simulink model "SPWM"  (R2022a)
settings: Solver=ode23  StartTime=0.0  StopTime=0.05  MaxStep=1e-5  RelTol=1e-3
libraries: simulink x2, spspowerguiLib x1
settings Model: Creator=123  LastModifiedBy=123

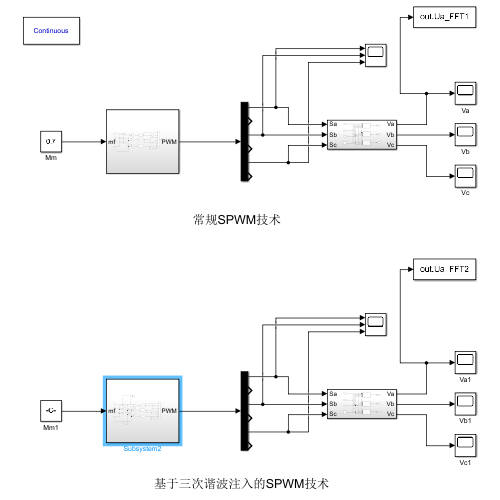
[thumbnail: Simulink's stored preview of the top-level diagram]
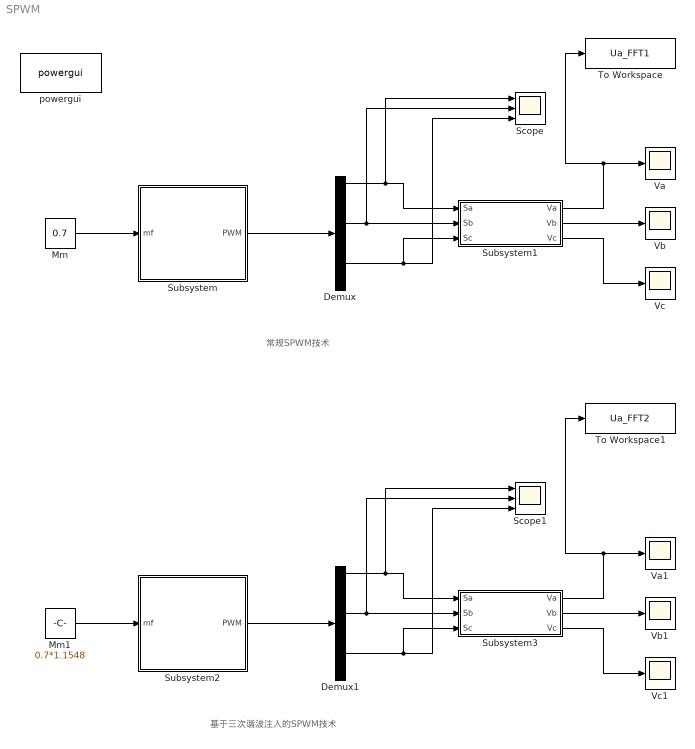
== system SPWM ==
  note: 基于三次谐波注入的SPWM技术
  note: 常规SPWM技术
  Demux : Demux  Outputs=6
  Demux1 : Demux  Outputs=6
  Mm : Constant  Value=0.7
  Mm1 : Constant  Value=0.7*1.1548
  Scope : Scope  NumInputPorts=3
  Scope1 : Scope  NumInputPorts=3
  Subsystem : Subsystem
  Subsystem1 : Subsystem
  Subsystem2 : Subsystem
  Subsystem3 : Subsystem
  To Workspace : ToWorkspace  VariableName=Ua_FFT1  SaveFormat=Structure With Time  SampleTime=1e-6
  To Workspace1 : ToWorkspace  VariableName=Ua_FFT2  SaveFormat=Structure With Time  SampleTime=1e-6
  Va : Scope
  Va1 : Scope
  Vb : Scope
  Vb1 : Scope
  Vc : Scope
  Vc1 : Scope
  powergui : spspowerguiLib/powergui  Priority=1  SimulationMode=Continuous  SampleTime=50e-6  frequency=60  Iterations=50  frequencyindice=60  Pbase=100e6  ErrMax=1e-4  UnitsV=kV  UnitsW=MW  buscounter=0  FunctionMessages=off  echomessages=off  EnableUseOfTLC=off  CurrentSourceSwitches=off  DisableSnubberDevices=off  DisableRonSwitches=off  DisableVfSwitches=off  DisplayEquations=off  AutomaticDiscreteSolvers=off  SolverType=Tustin/Backward Euler (TBE)  Interpol=off  ExternalGateDelay=off  methode=off  Ts=100  x0status=blocks  SPID=on  SwTol=0  HookPort=off  NonlinearTolerance=1e-4  nMaxIteration=100  ContinueOnMaxIteration=off  RestoreLinks=warning  ResistiveCurrentMeasurement=off  Frange=[0:2:500]  Ylog=off  Xlog=on  ShowGrid=off  save=off  variable=ZData  structure=0  ZoomFFT=off  StartTime=0.0  cycles=1  DisplayStyle=1  fundamental=60  FreqAxis=off  MaxFrequency=1000  frequencyindicesteady=1  RmsSteady=1  display=off
  wires:
  Mm/1 -> Subsystem/1(mf)
  Subsystem/1(PWM) -> Demux/1
  Demux/1 -> Scope/1, Subsystem1/1(Sa)
  Demux/3 -> Scope/2, Subsystem1/2(Sb)
  Demux/5 -> Scope/3, Subsystem1/3(Sc)
  Subsystem1/1(Va) -> Va/1, To Workspace/1
  Subsystem1/2(Vb) -> Vb/1
  Subsystem1/3(Vc) -> Vc/1
  Mm1/1 -> Subsystem2/1(mf)
  Subsystem2/1(PWM) -> Demux1/1
  Subsystem3/1(Va) -> Va1/1, To Workspace1/1
  Demux1/5 -> Scope1/3, Subsystem3/3(Sc)
  Subsystem3/3(Vc) -> Vc1/1
  Demux1/3 -> Scope1/2, Subsystem3/2(Sb)
  Subsystem3/2(Vb) -> Vb1/1
  Demux1/1 -> Scope1/1, Subsystem3/1(Sa)

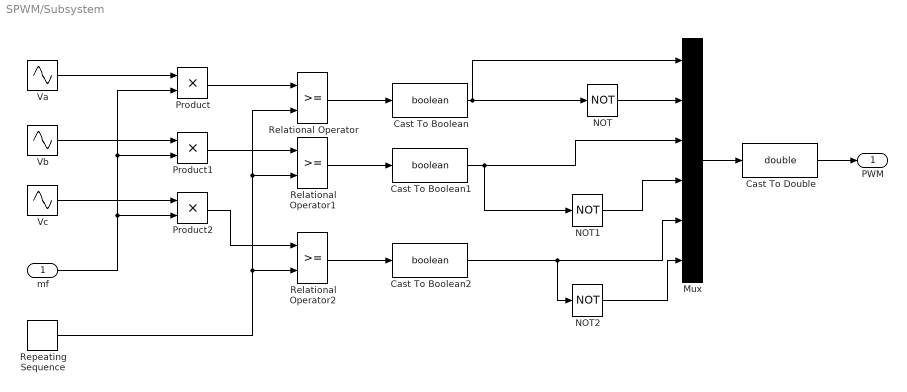
== system SPWM/Subsystem ==
  mf : Inport
  Cast To Boolean : DataTypeConversion  OutDataTypeStr=boolean  SaturateOnIntegerOverflow=off  RndMeth=Floor
  Cast To Boolean1 : DataTypeConversion  OutDataTypeStr=boolean  SaturateOnIntegerOverflow=off  RndMeth=Floor
  Cast To Boolean2 : DataTypeConversion  OutDataTypeStr=boolean  SaturateOnIntegerOverflow=off  RndMeth=Floor
  Cast To Double : DataTypeConversion  OutDataTypeStr=double  SaturateOnIntegerOverflow=off  RndMeth=Floor
  Mux : Mux  Inputs=6
  NOT : Logic  Operator=NOT  AllPortsSameDT=off  OutDataTypeStr=boolean
  NOT1 : Logic  Operator=NOT  AllPortsSameDT=off  OutDataTypeStr=boolean
  NOT2 : Logic  Operator=NOT  AllPortsSameDT=off  OutDataTypeStr=boolean
  Product : Product
  Product1 : Product
  Product2 : Product
  Relational Operator : RelationalOperator  OutDataTypeStr=boolean  RndMeth=Simplest  InputSameDT=off
  Relational Operator1 : RelationalOperator  OutDataTypeStr=boolean  RndMeth=Simplest  InputSameDT=off
  Relational Operator2 : RelationalOperator  OutDataTypeStr=boolean  RndMeth=Simplest  InputSameDT=off
  Repeating Sequence : simulink/Sources/Repeating Sequence  rep_seq_t=[0 0.00005 0.00015 0.0002]  rep_seq_y=[0 -1 1 0]
  Va : Sin  Frequency=2*50*pi  SampleTime=0
  Vb : Sin  Frequency=2*50*pi  Phase=-2/3*pi  SampleTime=0
  Vc : Sin  Frequency=2*50*pi  Phase=2/3*pi  SampleTime=0
  PWM : Outport
  wires:
  Va/1 -> Product/1
  mf/1 -> Product2/2, Product1/2, Product/2
  Vb/1 -> Product1/1
  Vc/1 -> Product2/1
  Product/1 -> Relational Operator/1
  Repeating Sequence/1 -> Relational Operator2/2, Relational Operator1/2, Relational Operator/2
  Product1/1 -> Relational Operator1/1
  Product2/1 -> Relational Operator2/1
  Relational Operator/1 -> Cast To Boolean/1
  Relational Operator2/1 -> Cast To Boolean2/1
  Relational Operator1/1 -> Cast To Boolean1/1
  Mux/1 -> Cast To Double/1
  Cast To Double/1 -> PWM/1
  Cast To Boolean/1 -> NOT/1, Mux/1
  NOT/1 -> Mux/2
  Cast To Boolean1/1 -> NOT1/1, Mux/3
  NOT1/1 -> Mux/4
  Cast To Boolean2/1 -> NOT2/1, Mux/5
  NOT2/1 -> Mux/6

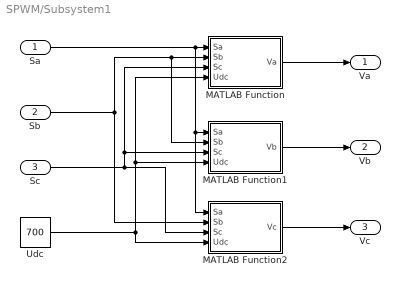
== system SPWM/Subsystem1 ==
  Sa : Inport
  Sb : Inport  Port=2
  Sc : Inport  Port=3
  MATLAB Function : MATLAB Function  TreatAsAtomicUnit=on
  MATLAB Function1 : MATLAB Function  TreatAsAtomicUnit=on
  MATLAB Function2 : MATLAB Function  TreatAsAtomicUnit=on
  Udc : Constant  Value=700
  Va : Outport
  Vb : Outport  Port=2
  Vc : Outport  Port=3
  wires:
  Sa/1 -> MATLAB Function1/1(Sa), MATLAB Function2/1(Sa), MATLAB Function/1(Sa)
  Sb/1 -> MATLAB Function2/2(Sb), MATLAB Function/2(Sb), MATLAB Function1/2(Sb)
  Sc/1 -> MATLAB Function2/3(Sc), MATLAB Function1/3(Sc), MATLAB Function/3(Sc)
  Udc/1 -> MATLAB Function2/4(Udc), MATLAB Function1/4(Udc), MATLAB Function/4(Udc)
  MATLAB Function2/1(Vc) -> Vc/1
  MATLAB Function1/1(Vb) -> Vb/1
  MATLAB Function/1(Va) -> Va/1

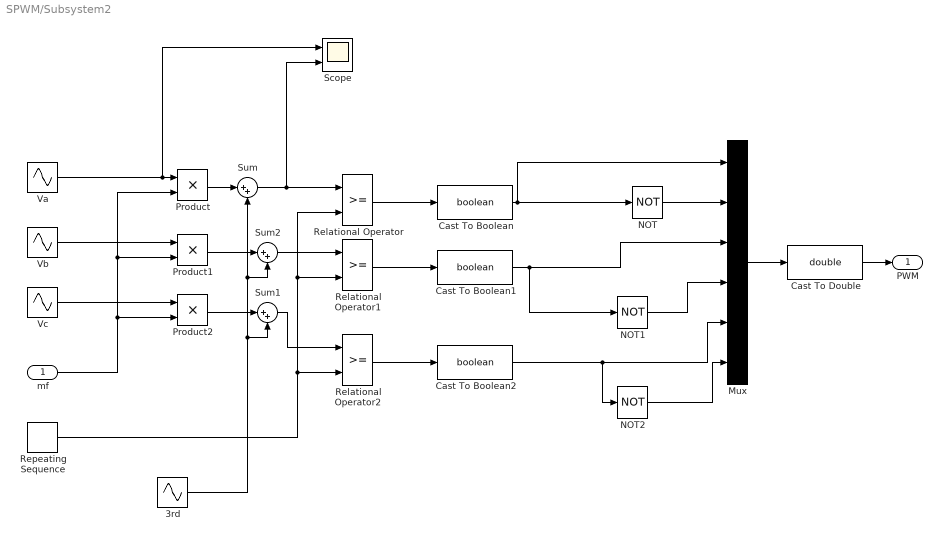
== system SPWM/Subsystem2 ==
  mf : Inport
  3rd : Sin  Amplitude=1*0.7*1.1548/6  Frequency=2*50*pi*3  SampleTime=0
  Cast To Boolean : DataTypeConversion  OutDataTypeStr=boolean  SaturateOnIntegerOverflow=off  RndMeth=Floor
  Cast To Boolean1 : DataTypeConversion  OutDataTypeStr=boolean  SaturateOnIntegerOverflow=off  RndMeth=Floor
  Cast To Boolean2 : DataTypeConversion  OutDataTypeStr=boolean  SaturateOnIntegerOverflow=off  RndMeth=Floor
  Cast To Double : DataTypeConversion  OutDataTypeStr=double  SaturateOnIntegerOverflow=off  RndMeth=Floor
  Mux : Mux  Inputs=6
  NOT : Logic  Operator=NOT  AllPortsSameDT=off  OutDataTypeStr=boolean
  NOT1 : Logic  Operator=NOT  AllPortsSameDT=off  OutDataTypeStr=boolean
  NOT2 : Logic  Operator=NOT  AllPortsSameDT=off  OutDataTypeStr=boolean
  Product : Product
  Product1 : Product
  Product2 : Product
  Relational Operator : RelationalOperator  OutDataTypeStr=boolean  RndMeth=Simplest  InputSameDT=off
  Relational Operator1 : RelationalOperator  OutDataTypeStr=boolean  RndMeth=Simplest  InputSameDT=off
  Relational Operator2 : RelationalOperator  OutDataTypeStr=boolean  RndMeth=Simplest  InputSameDT=off
  Repeating Sequence : simulink/Sources/Repeating Sequence  rep_seq_t=[0 0.00005 0.00015 0.0002]  rep_seq_y=[0 -1 1 0]
  Scope : Scope  NumInputPorts=2
  Sum : Sum  Inputs=|++
  Sum1 : Sum  Inputs=|++
  Sum2 : Sum  Inputs=|++
  Va : Sin  Frequency=2*50*pi  SampleTime=0
  Vb : Sin  Frequency=2*50*pi  Phase=-2/3*pi  SampleTime=0
  Vc : Sin  Frequency=2*50*pi  Phase=2/3*pi  SampleTime=0
  PWM : Outport
  wires:
  Va/1 -> Scope/1, Product/1
  mf/1 -> Product2/2, Product1/2, Product/2
  Vb/1 -> Product1/1
  Vc/1 -> Product2/1
  Repeating Sequence/1 -> Relational Operator2/2, Relational Operator1/2, Relational Operator/2
  Relational Operator/1 -> Cast To Boolean/1
  Relational Operator2/1 -> Cast To Boolean2/1
  Relational Operator1/1 -> Cast To Boolean1/1
  Mux/1 -> Cast To Double/1
  Cast To Double/1 -> PWM/1
  Cast To Boolean/1 -> NOT/1, Mux/1
  NOT/1 -> Mux/2
  Cast To Boolean1/1 -> NOT1/1, Mux/3
  NOT1/1 -> Mux/4
  Cast To Boolean2/1 -> NOT2/1, Mux/5
  NOT2/1 -> Mux/6
  Product/1 -> Sum/1
  3rd/1 -> Sum1/2, Sum2/2, Sum/2
  Sum/1 -> Scope/2, Relational Operator/1
  Product1/1 -> Sum2/1
  Product2/1 -> Sum1/1
  Sum2/1 -> Relational Operator1/1
  Sum1/1 -> Relational Operator2/1

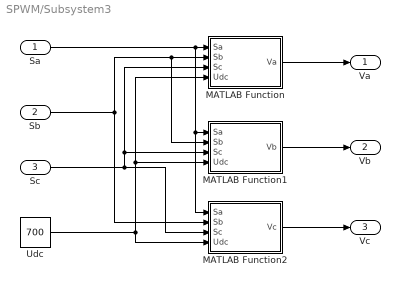
== system SPWM/Subsystem3 ==
  Sa : Inport
  Sb : Inport  Port=2
  Sc : Inport  Port=3
  MATLAB Function : MATLAB Function  TreatAsAtomicUnit=on
  MATLAB Function1 : MATLAB Function  TreatAsAtomicUnit=on
  MATLAB Function2 : MATLAB Function  TreatAsAtomicUnit=on
  Udc : Constant  Value=700
  Va : Outport
  Vb : Outport  Port=2
  Vc : Outport  Port=3
  wires:
  Sa/1 -> MATLAB Function1/1(Sa), MATLAB Function2/1(Sa), MATLAB Function/1(Sa)
  Sb/1 -> MATLAB Function2/2(Sb), MATLAB Function/2(Sb), MATLAB Function1/2(Sb)
  Sc/1 -> MATLAB Function2/3(Sc), MATLAB Function1/3(Sc), MATLAB Function/3(Sc)
  Udc/1 -> MATLAB Function2/4(Udc), MATLAB Function1/4(Udc), MATLAB Function/4(Udc)
  MATLAB Function2/1(Vc) -> Vc/1
  MATLAB Function1/1(Vb) -> Vb/1
  MATLAB Function/1(Va) -> Va/1

== matlab function SPWM/Subsystem1/MATLAB Function1 ==
  data: Sa input; Vb output; Sb input; Sc input; Udc input
function Vb = fcn(Sa,Sb,Sc,Udc)

Vb = Udc/3*(2*Sb - Sa - Sc);

== matlab function SPWM/Subsystem1/MATLAB Function ==
  data: Sa input; Va output; Sb input; Sc input; Udc input
function Va = fcn(Sa,Sb,Sc,Udc)

Va = Udc/3*(2*Sa - Sb - Sc);

== matlab function SPWM/Subsystem1/MATLAB Function2 ==
  data: Sa input; Vc output; Sb input; Sc input; Udc input
function Vc = fcn(Sa,Sb,Sc,Udc)

Vc = Udc/3*(2*Sc - Sb - Sa);

== matlab function SPWM/Subsystem3/MATLAB Function ==
  data: Sa input; Va output; Sb input; Sc input; Udc input
function Va = fcn(Sa,Sb,Sc,Udc)

Va = Udc/3*(2*Sa - Sb - Sc);

== matlab function SPWM/Subsystem3/MATLAB Function1 ==
  data: Sa input; Vb output; Sb input; Sc input; Udc input
function Vb = fcn(Sa,Sb,Sc,Udc)

Vb = Udc/3*(2*Sb - Sa - Sc);

== matlab function SPWM/Subsystem3/MATLAB Function2 ==
  data: Sa input; Vc output; Sb input; Sc input; Udc input
function Vc = fcn(Sa,Sb,Sc,Udc)

Vc = Udc/3*(2*Sc - Sb - Sa);
